simulink model "s_b16a4x512f"  (R2016b)
settings: Solver=VariableStepDiscrete  StartTime=0.0  StopTime=1  RelTol=1e-3
undefined symbols (not defined in the file): fft_stages, n_bits_ants, n_bits_xengs
libraries: xbsIndex_r4 x23057, casper_library_misc x150, xbsReplacements_r4 x9, casper_library_delays x8, xps_library x3
(part 31 of 210)

== system s_b16a4x512f/sys2/pack_out_skarab ==
  note: we must create a gap
      | between packets from
      | mutliple x-engines to allow
      | the buffers on the output switch
      | ports to drain and NIC card
      | to service the packets.
  note: if we become misaligned,
      | then we must flush the buffers
      | by reading one word, waiting "fifo_latency" clocks,
      | then reading another word until we get rb_done.
  note: the last packet
      | might be shorter!
  data_in : Inport
  valid_in : Inport  Port=2
  pkt_rdy : Inport  Port=3
  rb_done : Inport  Port=4
  timestamp : Inport  Port=5
  xeng_id : Inport  Port=6
  go : Inport  Port=7
  gap_size : Inport  Port=8
  AddSub1 : xbsIndex_r4/AddSub  mode=Subtraction  use_carryin=off  use_carryout=off  en=off  latency=1  precision=User Defined  arith_type=Unsigned  n_bits=vector_bits+1  bin_pt=0  quantization=Truncate  overflow=Saturate  use_behavioral_HDL=on  hw_selection=Fabric  pipelined=off  dbl_ovrd=off  block_type=addsub
  Concat : xbsIndex_r4/Concat  num_inputs=2  dbl_ovrd=off  block_type=concat
  Constant : xbsIndex_r4/Constant  const=0  gui_display_data_type=Boolean  arith_type=Boolean  n_bits=16  bin_pt=14  preci_type=Single  exp_width=8  frac_width=24  explicit_period=on  period=1  equ=P=C  opselect=C  inp2=PCIN>>17  opr=+  inp1=P  carry=CIN  dbl_ovrd=off  block_type=constant
  Constant1 : xbsIndex_r4/Constant  const=0  gui_display_data_type=Fixed-point  arith_type=Unsigned  n_bits=spead_lsw  bin_pt=0  preci_type=Single  exp_width=8  frac_width=24  explicit_period=on  period=1  equ=P=C  opselect=C  inp2=PCIN>>17  opr=+  inp1=P  carry=CIN  dbl_ovrd=off  block_type=constant
  Constant15 : xbsIndex_r4/Constant  const=pkt_len  gui_display_data_type=Fixed-point  arith_type=Unsigned  n_bits=vector_bits+1  bin_pt=0  preci_type=Single  exp_width=8  frac_width=24  explicit_period=on  period=1  equ=P=C  opselect=C  inp2=PCIN>>17  opr=+  inp1=P  carry=CIN  dbl_ovrd=off  block_type=constant
  Constant2 : xbsIndex_r4/Constant  const=(vector_len)-1  gui_display_data_type=Fixed-point  arith_type=Unsigned  n_bits=vector_bits+1  bin_pt=0  preci_type=Single  exp_width=8  frac_width=24  explicit_period=on  period=1  equ=P=C  opselect=C  inp2=PCIN>>17  opr=+  inp1=P  carry=CIN  dbl_ovrd=off  block_type=constant
  Constant3 : xbsIndex_r4/Constant  const=vector_len  gui_display_data_type=Fixed-point  arith_type=Unsigned  n_bits=vector_bits+1  bin_pt=0  preci_type=Single  exp_width=8  frac_width=24  explicit_period=on  period=1  equ=P=C  opselect=C  inp2=PCIN>>17  opr=+  inp1=P  carry=CIN  dbl_ovrd=off  block_type=constant
  Constant4 : xbsIndex_r4/Constant  const=0  gui_display_data_type=Boolean  arith_type=Boolean  n_bits=16  bin_pt=14  preci_type=Single  exp_width=8  frac_width=24  explicit_period=on  period=1  equ=P=C  opselect=C  inp2=PCIN>>17  opr=+  inp1=P  carry=CIN  dbl_ovrd=off  block_type=constant
  Constant6 : xbsIndex_r4/Constant  const=heap_len  gui_display_data_type=Fixed-point  arith_type=Unsigned  n_bits=spead_lsw  bin_pt=0  preci_type=Single  exp_width=8  frac_width=24  explicit_period=on  period=1  equ=P=C  opselect=C  inp2=PCIN>>17  opr=+  inp1=P  carry=CIN  dbl_ovrd=off  block_type=constant
  Constant7 : xbsIndex_r4/Constant  const=pkt_len-1  gui_display_data_type=Fixed-point  arith_type=Unsigned  n_bits=pkt_bits  bin_pt=0  preci_type=Single  exp_width=8  frac_width=24  explicit_period=on  period=1  equ=P=C  opselect=C  inp2=PCIN>>17  opr=+  inp1=P  carry=CIN  dbl_ovrd=off  block_type=constant
  Constant8 : xbsIndex_r4/Constant  const=1  gui_display_data_type=Fixed-point  arith_type=Unsigned  n_bits=ceil(log2(fifo_latency))+1  bin_pt=0  preci_type=Single  exp_width=8  frac_width=24  explicit_period=on  period=1  equ=P=C  opselect=C  inp2=PCIN>>17  opr=+  inp1=P  carry=CIN  dbl_ovrd=off  block_type=constant
  Convert{,1..4,6} (6 alike) : xbsIndex_r4/Convert  gui_display_data_type=Fixed-point  arith_type=Unsigned  n_bits=spead_lsw  bin_pt=0  float_type=Single  exp_bits=8  fraction_bits=24  quantization=Truncate  overflow=Wrap  en=off  latency=0  pipeline=off  dbl_ovrd=off  block_type=convert
      settings: block_version=11.4
  Counter1 : xbsIndex_r4/Counter  cnt_type=Free Running  cnt_to=1023  operation=Up  start_count=0  cnt_by_val=1  arith_type=Unsigned  n_bits=vector_bits+1  bin_pt=0  load_pin=off  rst=on  en=on  explicit_period=on  period=1  use_behavioral_HDL=off  implementation=Fabric  use_rpm=on  dbl_ovrd=off  block_type=counter
      settings: xl_area=[0, 0, 0, 0, 0, 0, 0]
  Delay{,3,10..17} (10 alike) : xbsIndex_r4/Delay  rst=off  infoeditControl=Selection of Reset will increase slice count due to use of real FFs and instead of SRLs  en=off  latency=1  reg_retiming=on  dbl_ovrd=off  block_type=delay
      settings: block_version=11.4
  Delay1 : xbsIndex_r4/Delay  rst=off  infoeditControl=Selection of Reset will increase slice count due to use of real FFs and instead of SRLs  en=on  latency=1  reg_retiming=on  dbl_ovrd=off  block_type=delay
  Delay2 : xbsIndex_r4/Delay  rst=off  infoeditControl=Selection of Reset will increase slice count due to use of real FFs and instead of SRLs  en=off  latency=fifo_latency  reg_retiming=on  dbl_ovrd=off  block_type=delay
      settings: block_version=11.4
  Delay4 : xbsIndex_r4/Delay  rst=off  infoeditControl=Selection of Reset will increase slice count due to use of real FFs and instead of SRLs  en=off  latency=fifo_latency  reg_retiming=on  dbl_ovrd=off  block_type=delay
      settings: block_version=11.4
  Delay5 : xbsIndex_r4/Delay  rst=off  infoeditControl=Selection of Reset will increase slice count due to use of real FFs and instead of SRLs  en=on  latency=1  reg_retiming=on  dbl_ovrd=off  block_type=delay
  Delay7 : xbsIndex_r4/Delay  rst=on  infoeditControl=Selection of Reset will increase slice count due to use of real FFs and instead of SRLs  en=on  latency=1  reg_retiming=on  dbl_ovrd=off  block_type=delay
  Delay8 : xbsIndex_r4/Delay  rst=on  infoeditControl=Selection of Reset will increase slice count due to use of real FFs and instead of SRLs  en=on  latency=1  reg_retiming=on  dbl_ovrd=off  block_type=delay
  Delay9 : xbsIndex_r4/Delay  rst=on  infoeditControl=Selection of Reset will increase slice count due to use of real FFs and instead of SRLs  en=on  latency=1  reg_retiming=on  dbl_ovrd=off  block_type=delay
  Gateway Out{1..21} (21 alike) : xbsIndex_r4/Gateway Out  inherit_from_input=off  hdl_port=off  rows=1  columns=1  UseAsDAC=off  DACChannel='1'  interface=None  automatic_assignment=on  address_offset=hex2dec('00')  intf_name=''  intf_description=''  timing_constraint=None  locs_specified=off  LOCs={}  io_standard={}  block_type=gatewayout
      settings: xl_area=[0, 0, 0, 0, 0, 0, 0]  block_version=10.1.3
  Inverter{1..4} (4 alike) : xbsIndex_r4/Inverter  en=off  latency=0  dbl_ovrd=off  block_type=inv
      settings: block_version=11.4
  Logical{1,3..5,13..14} (6 alike) : xbsIndex_r4/Logical  logical_function=OR  inputs=2  en=off  latency=0  precision=Full  arith_type=Unsigned  n_bits=8  bin_pt=2  align_bp=on  dbl_ovrd=off  block_type=logical
      settings: xl_area=[0, 0, 0, 0, 0, 0, 0]
  Logical{2,8..12,15} (7 alike) : xbsIndex_r4/Logical  logical_function=AND  inputs=2  en=off  latency=0  precision=Full  arith_type=Unsigned  n_bits=8  bin_pt=2  align_bp=on  dbl_ovrd=off  block_type=logical
      settings: xl_area=[0, 0, 0, 0, 0, 0, 0]
  Logical6 : xbsIndex_r4/Logical  logical_function=AND  inputs=2  en=off  latency=1  precision=Full  arith_type=Unsigned  n_bits=8  bin_pt=2  align_bp=on  dbl_ovrd=off  block_type=logical
      settings: xl_area=[0, 0, 0, 0, 0, 0, 0]
  Logical7 : xbsIndex_r4/Logical  logical_function=XOR  inputs=2  en=off  latency=0  precision=Full  arith_type=Unsigned  n_bits=8  bin_pt=2  align_bp=on  dbl_ovrd=off  block_type=logical
      settings: xl_area=[0, 0, 0, 0, 0, 0, 0]
  Mux1 : xbsIndex_r4/Mux  inputs=2  en=off  latency=1  precision=Full  arith_type="Signed  (2's comp)"  n_bits=8  bin_pt=2  quantization=Truncate  overflow=Wrap  dbl_ovrd=off  block_type=mux
      settings: xl_area=[0, 0, 0, 0, 0, 0, 0]
  Reinterpret : xbsIndex_r4/Reinterpret  force_arith_type=on  arith_type=Unsigned  force_bin_pt=on  bin_pt=0  block_type=reinterpret
      settings: infoedit="Changes signal type without altering the binary representation.   You can changed the signal between signed and unsigned, and relocate the binary point.<br><br>Hardware notes: In hardware this block costs nothing.<br><br>Example:  Suppose the input is 6 bits wide, signed, with 2 fractional bits, and the output is forced to unsigned with 0 fractional bits.  Then an input of -2.0 (1110.00 in binary 2's complement) becomes an output of 56 (111000 in binary)."
  Relational1 : xbsIndex_r4/Relational  mode=a=b  op_type=Bool  en=off  latency=0  dbl_ovrd=off  block_type=relational
      settings: xl_area=[0, 0, 0, 0, 0, 0, 0]  block_version=10.1.3
  Relational2 : xbsIndex_r4/Relational  mode=a<b  op_type=Bool  en=off  latency=0  dbl_ovrd=off  block_type=relational
      settings: xl_area=[0, 0, 0, 0, 0, 0, 0]  block_version=10.1.3
  Relational4 : xbsIndex_r4/Relational  mode=a=b  op_type=Bool  en=off  latency=0  dbl_ovrd=off  block_type=relational
      settings: xl_area=[0, 0, 0, 0, 0, 0, 0]  block_version=10.1.3
  Relational5 : xbsIndex_r4/Relational  mode=a=b  op_type=Bool  en=off  latency=0  dbl_ovrd=off  block_type=relational
      settings: xl_area=[0, 0, 0, 0, 0, 0, 0]  block_version=10.1.3
  Shift1 : xbsIndex_r4/Shift  shift_dir=Left  shift_bits=n_bits_word_size  en=off  latency=0  precision=Full  arith_type="Signed  (2's comp)"  n_bits=16  bin_pt=14  quantization=Truncate  overflow=Wrap  dbl_ovrd=off  block_type=shift
  Shift2 : xbsIndex_r4/Shift  shift_dir=Left  shift_bits=n_bits_chans  en=off  latency=0  precision=Full  arith_type="Signed  (2's comp)"  n_bits=16  bin_pt=14  quantization=Truncate  overflow=Wrap  dbl_ovrd=off  block_type=shift
  Slice : xbsIndex_r4/Slice  nbits=pkt_bits  boolean_output=off  mode=Lower Bit Location + Width  bit1=0  base1=MSB of Input  bit0=0  base0=LSB of Input  dbl_ovrd=off  block_type=slice
  Slice1 : xbsIndex_r4/Slice  nbits=1  boolean_output=off  mode=Two Bit Locations  bit1=0  base1=MSB of Input  bit0=n_bits_timestamp_padding  base0=LSB of Input  dbl_ovrd=off  block_type=slice
  edge_detect : Subsystem  AncestorBlock=casper_library_misc/edge_detect  mask(edge_detect){edge=Rising, polarity=Active High, x_in=[0 0.08 0.08 0.16 0.16 0.24 0.24 0.32 0.32 0.4], y_in=[-1 -1  1  1  1  1  1  1  1  1], x_out=[0.6 0.68 0.68 0.76 0.76 0.84 0.84 0.92 0.92 1], y_out=[-1 -1  1  1 -1 -1 -1 -1 -1 -1]}
      mask prompts: edge "Edge Type"; polarity "Output Polarity"; x_in "Input X Positions"; y_in "Input Y Positions"; x_out "Output X Positions"; y_out "Output Y Positions"
      mask help: Output is active for one-cycle after each edge of the specified type (i.e. rising, falling or both).
      mask init: same as s_b16a4x512f/edge_detect
      settings: AttributesFormatString=|
      | rising edges
      | active high
      mask Help: Output is active for one-cycle after each edge of the specified type (i.e. rising, falling, or both).  Latency is zero.
      mask TypeOptions edge: Rising | Falling | Both
      mask TypeOptions polarity: Active High | Active Low
      mask Display:
      | plot(x_in_num,0.5+y_in_num*0.2);
      | plot(x_out_num,0.5+y_out_num*0.2);
  edge_detect1 : Subsystem  AncestorBlock=casper_library_misc/edge_detect  mask(edge_detect){edge=Rising, polarity=Active High, x_in=[0 0.08 0.08 0.16 0.16 0.24 0.24 0.32 0.32 0.4], y_in=[-1 -1  1  1  1  1  1  1  1  1], x_out=[0.6 0.68 0.68 0.76 0.76 0.84 0.84 0.92 0.92 1], y_out=[-1 -1  1  1 -1 -1 -1 -1 -1 -1]}
      mask prompts: edge "Edge Type"; polarity "Output Polarity"; x_in "Input X Positions"; y_in "Input Y Positions"; x_out "Output X Positions"; y_out "Output Y Positions"
      mask help: Output is active for one-cycle after each edge of the specified type (i.e. rising, falling or both).
      mask init: same as s_b16a4x512f/edge_detect
      settings: AttributesFormatString=|
      | rising edges
      | active high
      mask Help: Output is active for one-cycle after each edge of the specified type (i.e. rising, falling, or both).  Latency is zero.
      mask TypeOptions edge: Rising | Falling | Both
      mask TypeOptions polarity: Active High | Active Low
      mask Display:
      | plot(x_in_num,0.5+y_in_num*0.2);
      | plot(x_out_num,0.5+y_out_num*0.2);
  edge_detect2 : Subsystem  AncestorBlock=casper_library_misc/edge_detect  mask(edge_detect){edge=Rising, polarity=Active High, x_in=[0 0.08 0.08 0.16 0.16 0.24 0.24 0.32 0.32 0.4], y_in=[-1 -1  1  1  1  1  1  1  1  1], x_out=[0.6 0.68 0.68 0.76 0.76 0.84 0.84 0.92 0.92 1], y_out=[-1 -1  1  1 -1 -1 -1 -1 -1 -1]}
      mask prompts: edge "Edge Type"; polarity "Output Polarity"; x_in "Input X Positions"; y_in "Input Y Positions"; x_out "Output X Positions"; y_out "Output Y Positions"
      mask help: Output is active for one-cycle after each edge of the specified type (i.e. rising, falling or both).
      mask init: same as s_b16a4x512f/edge_detect
      settings: AttributesFormatString=|
      | rising edges
      | active high
      mask Help: Output is active for one-cycle after each edge of the specified type (i.e. rising, falling, or both).  Latency is zero.
      mask TypeOptions edge: Rising | Falling | Both
      mask TypeOptions polarity: Active High | Active Low
      mask Display:
      | plot(x_in_num,0.5+y_in_num*0.2);
      | plot(x_out_num,0.5+y_out_num*0.2);
  edge_detect3 : Subsystem  AncestorBlock=casper_library_misc/edge_detect  mask(edge_detect){edge=Rising, polarity=Active High, x_in=[0 0.08 0.08 0.16 0.16 0.24 0.24 0.32 0.32 0.4], y_in=[-1 -1  1  1  1  1  1  1  1  1], x_out=[0.6 0.68 0.68 0.76 0.76 0.84 0.84 0.92 0.92 1], y_out=[-1 -1  1  1 -1 -1 -1 -1 -1 -1]}
      mask prompts: edge "Edge Type"; polarity "Output Polarity"; x_in "Input X Positions"; y_in "Input Y Positions"; x_out "Output X Positions"; y_out "Output Y Positions"
      mask help: Output is active for one-cycle after each edge of the specified type (i.e. rising, falling or both).
      mask init: same as s_b16a4x512f/edge_detect
      settings: AttributesFormatString=|
      | rising edges
      | active high
      mask Help: Output is active for one-cycle after each edge of the specified type (i.e. rising, falling, or both).  Latency is zero.
      mask TypeOptions edge: Rising | Falling | Both
      mask TypeOptions polarity: Active High | Active Low
      mask Display:
      | plot(x_in_num,0.5+y_in_num*0.2);
      | plot(x_out_num,0.5+y_out_num*0.2);
  edge_detect4 : Subsystem  AncestorBlock=casper_library_misc/edge_detect  mask(edge_detect){edge=Rising, polarity=Active High, x_in=[0 0.08 0.08 0.16 0.16 0.24 0.24 0.32 0.32 0.4], y_in=[-1 -1  1  1  1  1  1  1  1  1], x_out=[0.6 0.68 0.68 0.76 0.76 0.84 0.84 0.92 0.92 1], y_out=[-1 -1  1  1 -1 -1 -1 -1 -1 -1]}
      mask prompts: edge "Edge Type"; polarity "Output Polarity"; x_in "Input X Positions"; y_in "Input Y Positions"; x_out "Output X Positions"; y_out "Output Y Positions"
      mask help: Output is active for one-cycle after each edge of the specified type (i.e. rising, falling or both).
      mask init: same as s_b16a4x512f/edge_detect
      settings: AttributesFormatString=|
      | rising edges
      | active high
      mask Help: Output is active for one-cycle after each edge of the specified type (i.e. rising, falling, or both).  Latency is zero.
      mask TypeOptions edge: Rising | Falling | Both
      mask TypeOptions polarity: Active High | Active Low
      mask Display:
      | plot(x_in_num,0.5+y_in_num*0.2);
      | plot(x_out_num,0.5+y_out_num*0.2);
  gap_creator : xbsIndex_r4/Counter  cnt_type=Free Running  cnt_to=Inf  operation=Up  start_count=0  cnt_by_val=1  arith_type=Unsigned  n_bits=n_bits_max_gap  bin_pt=0  load_pin=off  rst=on  en=on  explicit_period=on  period=1  use_behavioral_HDL=off  implementation=Fabric  dbl_ovrd=off  block_type=counter
  gap_done : xbsIndex_r4/Relational  mode=a<b  op_type=Bool  en=off  latency=1  dbl_ovrd=off  block_type=relational
  hdr_check : Scope  NumInputPorts=5
  hdr_check1 : Scope  NumInputPorts=5
  pack_xeng : Subsystem  Tag=casper:spead_pack  AncestorBlock=casper_library_communications/spead_pack  mask(pkt_pack_mask){max_pkt_len_bits=8, header_ids=0x1600, 0x4103, header_ind_ids=0x1800, spead_msw=64, spead_lsw=48, spead_version=4, bytes_per_word=8}
      mask prompts: max_pkt_len_bits "Max pkt length, 2^? 64-bit words"; header_ids "SPEAD direct address IDs (decimal)"; header_ind_ids "SPEAD indirect address IDs (decimal)"; spead_msw "SPEAD Flavour (MSw)"; spead_lsw "SPEAD Flavour (LSw)"; spead_version "SPEAD version"; bytes_per_word "Word size, in bytes"
      mask help:
      | This block generates SPEAD-compliant packets from a datastream.
      |
      | Packets are created with a fixed header followed by a number of 64-bit items.
      |
      | Requires a 64-bit data stream.
      |
      | The data_ready signal is one cycle BEFORE valid data! Does not have to be with a valid signal either.
      mask init:
      | % if floor(log2(bytes_per_word)) ~= log2(bytes_per_word)
      | %     error('Bytes per word should be a power of two.');
      | % end
      | % 
      | % spead_pack_init(gcb)
  packetise_output : Scope  NumInputPorts=11
  payload_cnt4 : xbsIndex_r4/Counter  cnt_type=Count Limited  cnt_to=max((fifo_latency + 1),2)  operation=Up  start_count=0  cnt_by_val=1  arith_type=Unsigned  n_bits=ceil(log2(fifo_latency))+1  bin_pt=0  load_pin=off  rst=on  en=on  explicit_period=on  period=1  use_behavioral_HDL=off  implementation=Fabric  use_rpm=on  dbl_ovrd=off  block_type=counter
      settings: xl_area=[0, 0, 0, 0, 0, 0, 0]
  data_out : Outport
  valid_out : Outport  Port=2
  eof : Outport  Port=3
  err : Outport  Port=4
  fetch : Outport  Port=5
  pkt_ready : Outport  Port=6
  wires:
  edge_detect4/1(out) -> gap_creator/1
  Convert6/1 -> Shift2/1
  Constant1/1 -> pack_xeng/10(hdr8_0x1800)
  Convert2/1 -> [heap_cnt]
  Concat/1 -> Convert2/1
  [xeng_id] -> Concat/2
  Slice1/1 -> Concat/1
  [timestamp] -> Slice1/1
  gap_size/1 -> [gap_size]
  Delay13/1 -> pack_xeng/9(hdr6_0x4103_DIR)
  [freq_offset] -> Delay13/1
  Shift2/1 -> [freq_offset]
  [xeng_id] -> Convert6/1
  Convert4/1 -> Delay16/1
  [gap_size] -> gap_done/2
  pack_xeng/3(eof) -> Logical3/1
  Logical3/1 -> eof/1
  Gateway Out15/1 -> packetise_output/7
  [end_of_vector] -> Logical5/1
  Gateway Out9/1 -> packetise_output/6
  Gateway Out14/1 -> packetise_output/5
  Gateway Out6/1 -> packetise_output/4
  Gateway Out8/1 -> packetise_output/3
  Gateway Out1/1 -> packetise_output/2
  Gateway Out7/1 -> packetise_output/1
  Logical5/1 -> [eof]
  Logical2/1 -> [rb_done]
  xeng_id/1 -> [xeng_id]
  Reinterpret/1 -> [data_input]
  Gateway Out11/1 -> packetise_output/8
  Slice/1 -> Relational1/1
  Counter1/1 -> [vector_position], Slice/1, Relational5/1
  timestamp/1 -> Delay5/1
  Delay5/1 -> [timestamp]
  [vector_start] -> Delay5/2
  Constant2/1 -> Relational5/2
  Relational5/1 -> [end_of_vector]
  data_in/1 -> Reinterpret/1, [raw_data_input]
  valid_in/1 -> Logical2/1, [valid_input]
  pkt_rdy/1 -> [pkt_rdy]
  rb_done/1 -> Logical2/2
  Gateway Out18/1 -> packetise_output/9
  Gateway Out17/1 -> packetise_output/10
  [valid_input] -> [valid_output]
  [fetch_pld] -> Counter1/2
  [vector_start] -> Counter1/1
  Constant7/1 -> Relational1/2
  Relational1/1 -> Logical5/2
  [fetch_pld] -> Gateway Out6/1
  [busy] -> Gateway Out15/1
  [valid_output] -> Gateway Out1/1
  [busy_pkt] -> Gateway Out9/1
  [raw_data_input] -> Gateway Out7/1
  [vector_position] -> Gateway Out11/1
  pack_xeng/1(data_out) -> data_out/1, [data_out]
  [vector_position] -> Delay1/1
  Delay1/1 -> AddSub1/2, Delay17/1
  [get_a_pkt] -> Delay1/2
  [rb_done] -> Logical7/1
  [end_of_vector] -> Delay2/1
  Delay17/1 -> Convert/1
  Convert/1 -> Shift1/1
  [vector_start] -> Logical4/1
  Logical4/1 -> Delay4/1
  [go] -> Logical8/1
  Logical8/1 -> Delay3/1
  Delay7/1 -> [busy], edge_detect/1(in)
  edge_detect/1(out) -> [vector_start]
  Inverter2/1 -> Logical10/1
  Logical10/1 -> Delay7/1, Delay7/3
  [end_of_vector] -> Logical1/2
  [go] -> Delay/1
  edge_detect1/1(out) -> Logical10/2
  [busy] -> Inverter2/1
  Delay/1 -> edge_detect1/1(in)
  Delay2/1 -> Logical7/2
  [get_a_pkt] -> Inverter1/1
  Delay3/1 -> Logical4/2
  Delay4/1 -> Delay8/1, Delay8/3
  edge_detect2/1(out) -> [get_a_pkt]
  Delay8/1 -> [busy_pkt], edge_detect2/1(in)
  [eof] -> Delay8/2
  [busy] -> Logical8/2
  Inverter1/1 -> Logical9/1
  Logical9/1 -> [fetch_pld]
  [eof] -> Gateway Out18/1
  [pkt_rdy] -> Gateway Out17/1
  Logical7/1 -> Delay9/1, Delay9/3, [err]
  [rb_done] -> Logical12/2
  payload_cnt4/1 -> Relational4/2
  Constant8/1 -> Relational4/1
  Delay9/1 -> payload_cnt4/2, [flushing]
  Relational4/1 -> [stutter_flush]
  Logical1/1 -> Delay7/2
  [err] -> Logical1/1
  [valid_output] -> Logical11/1
  Inverter3/1 -> Logical11/2, Logical15/2
  [flushing] -> Inverter3/1
  Logical12/1 -> Delay9/2, payload_cnt4/1
  [flushing] -> Logical12/1
  Logical13/1 -> fetch/1
  [fetch_pld] -> Logical13/1
  [stutter_flush] -> Logical13/2
  [data_out] -> Gateway Out2/1
  [vector_start] -> Gateway Out3/1
  [heap_cnt] -> Gateway Out4/1
  [heap_offset] -> Gateway Out5/1
  Gateway Out2/1 -> hdr_check/1
  Gateway Out3/1 -> hdr_check/2
  Gateway Out4/1 -> hdr_check/3
  Gateway Out5/1 -> hdr_check/4
  Constant15/1 -> Relational2/2, Mux1/2
  Mux1/1 -> Convert1/1
  Relational2/1 -> Mux1/1
  Constant3/1 -> AddSub1/1
  AddSub1/1 -> Mux1/3, Relational2/1
  Convert1/1 -> [pld_len]
  Shift1/1 -> [heap_offset]
  Gateway Out10/1 -> hdr_check/5
  [pld_len] -> Gateway Out10/1
  gap_creator/1 -> gap_done/1, [gap_count]
  go/1 -> [go]
  gap_done/1 -> Inverter4/1, gap_creator/2
  Inverter4/1 -> Logical6/1
  [pkt_rdy] -> Logical6/2
  Logical6/1 -> pkt_ready/1
  [eof] -> edge_detect4/1(in)
  Gateway Out16/1 -> packetise_output/11
  [gap_count] -> Gateway Out16/1
  [data_input] -> Delay11/1
  [heap_cnt] -> Convert3/1
  [heap_offset] -> Delay14/1
  Logical11/1 -> Delay10/1
  pack_xeng/2(valid_out) -> valid_out/1
  [pld_len] -> Delay15/1
  Logical14/1 -> Logical3/2, err/1
  pack_xeng/4(data_overflow) -> [data_overflow], Logical14/2
  [err] -> Logical14/1
  [valid_output] -> Logical15/1
  edge_detect3/1(out) -> pack_xeng/1(data256_ready)
  Logical15/1 -> edge_detect3/1(in)
  Delay10/1 -> pack_xeng/2(data256_valid)
  Delay11/1 -> pack_xeng/3(data256)
  Delay12/1 -> pack_xeng/4(hdr_heap_id)
  Constant6/1 -> pack_xeng/5(hdr_heap_size)
  Delay14/1 -> pack_xeng/6(hdr_heap_offset)
  Delay15/1 -> pack_xeng/7(hdr_pkt_len_words)
  Delay16/1 -> pack_xeng/8(hdr5_0x1600_DIR)
  Gateway Out20/1 -> hdr_check1/4
  Gateway Out12/1 -> hdr_check1/1
  Gateway Out19/1 -> hdr_check1/3
  Gateway Out21/1 -> hdr_check1/5
  Gateway Out13/1 -> hdr_check1/2
  [valid_input] -> Gateway Out12/1
  [rb_done] -> Gateway Out13/1
  [end_of_vector] -> Gateway Out19/1
  [err] -> Gateway Out20/1
  [data_overflow] -> Gateway Out21/1
  [busy_pkt] -> Logical9/2
  Constant/1 -> Gateway Out8/1
  Constant4/1 -> Gateway Out14/1
  Convert3/1 -> Delay12/1
  [timestamp] -> Convert4/1

== system s_b16a4x512f/sys2/pipeline ==
  d : Inport
  Register0 : xbsIndex_r4/Register  init=0  rst=off  en=off  dbl_ovrd=off  block_type=register
      settings: block_version=11.4
  Register1 : xbsIndex_r4/Register  init=0  rst=off  en=off  dbl_ovrd=off  block_type=register
      settings: block_version=11.4
  q : Outport
  wires:
  Register0/1 -> Register1/1
  d/1 -> Register0/1
  Register1/1 -> q/1

== system s_b16a4x512f/sys2/pipeline1 ==
  d : Inport
  Register0 : xbsIndex_r4/Register  init=0  rst=off  en=off  dbl_ovrd=off  block_type=register
      settings: block_version=11.4
  Register1 : xbsIndex_r4/Register  init=0  rst=off  en=off  dbl_ovrd=off  block_type=register
      settings: block_version=11.4
  q : Outport
  wires:
  Register1/1 -> q/1
  d/1 -> Register0/1
  Register0/1 -> Register1/1

== system s_b16a4x512f/sys2/pipeline10 ==
  d : Inport
  Register0 : xbsIndex_r4/Register  init=0  rst=off  en=off  dbl_ovrd=off  block_type=register
      settings: block_version=11.4
  Register1 : xbsIndex_r4/Register  init=0  rst=off  en=off  dbl_ovrd=off  block_type=register
      settings: block_version=11.4
  q : Outport
  wires:
  Register0/1 -> Register1/1
  d/1 -> Register0/1
  Register1/1 -> q/1

== system s_b16a4x512f/sys2/pipeline11 ==
  d : Inport
  Register0 : xbsIndex_r4/Register  init=0  rst=off  en=off  dbl_ovrd=off  block_type=register
      settings: block_version=11.4
  Register1 : xbsIndex_r4/Register  init=0  rst=off  en=off  dbl_ovrd=off  block_type=register
      settings: block_version=11.4
  q : Outport
  wires:
  Register1/1 -> q/1
  d/1 -> Register0/1
  Register0/1 -> Register1/1

== system s_b16a4x512f/sys2/pipeline12 ==
  d : Inport
  Register0 : xbsIndex_r4/Register  init=0  rst=off  en=off  dbl_ovrd=off  block_type=register
      settings: block_version=11.4
  Register1 : xbsIndex_r4/Register  init=0  rst=off  en=off  dbl_ovrd=off  block_type=register
      settings: block_version=11.4
  q : Outport
  wires:
  Register0/1 -> Register1/1
  d/1 -> Register0/1
  Register1/1 -> q/1

== system s_b16a4x512f/sys2/pipeline13 ==
  d : Inport
  Register0 : xbsIndex_r4/Register  init=0  rst=off  en=off  dbl_ovrd=off  block_type=register
      settings: block_version=11.4
  Register1 : xbsIndex_r4/Register  init=0  rst=off  en=off  dbl_ovrd=off  block_type=register
      settings: block_version=11.4
  q : Outport
  wires:
  Register1/1 -> q/1
  d/1 -> Register0/1
  Register0/1 -> Register1/1

== system s_b16a4x512f/sys2/pipeline2 ==
  d : Inport
  Register0 : xbsIndex_r4/Register  init=0  rst=off  en=off  dbl_ovrd=off  block_type=register
      settings: block_version=11.4
  Register1 : xbsIndex_r4/Register  init=0  rst=off  en=off  dbl_ovrd=off  block_type=register
      settings: block_version=11.4
  q : Outport
  wires:
  Register0/1 -> Register1/1
  d/1 -> Register0/1
  Register1/1 -> q/1

== system s_b16a4x512f/sys2/pipeline3 ==
  d : Inport
  Register0 : xbsIndex_r4/Register  init=0  rst=off  en=off  dbl_ovrd=off  block_type=register
      settings: block_version=11.4
  Register1 : xbsIndex_r4/Register  init=0  rst=off  en=off  dbl_ovrd=off  block_type=register
      settings: block_version=11.4
  q : Outport
  wires:
  Register1/1 -> q/1
  d/1 -> Register0/1
  Register0/1 -> Register1/1

== system s_b16a4x512f/sys2/pipeline4 ==
  d : Inport
  Register0 : xbsIndex_r4/Register  init=0  rst=off  en=off  dbl_ovrd=off  block_type=register
      settings: block_version=11.4
  Register1 : xbsIndex_r4/Register  init=0  rst=off  en=off  dbl_ovrd=off  block_type=register
      settings: block_version=11.4
  q : Outport
  wires:
  Register1/1 -> q/1
  d/1 -> Register0/1
  Register0/1 -> Register1/1

== system s_b16a4x512f/sys2/pipeline5 ==
  d : Inport
  Register0 : xbsIndex_r4/Register  init=0  rst=off  en=off  dbl_ovrd=off  block_type=register
      settings: block_version=11.4
  Register1 : xbsIndex_r4/Register  init=0  rst=off  en=off  dbl_ovrd=off  block_type=register
      settings: block_version=11.4
  q : Outport
  wires:
  Register0/1 -> Register1/1
  d/1 -> Register0/1
  Register1/1 -> q/1

== system s_b16a4x512f/sys2/pipeline6 ==
  d : Inport
  Register0 : xbsIndex_r4/Register  init=0  rst=off  en=off  dbl_ovrd=off  block_type=register
      settings: block_version=11.4
  Register1 : xbsIndex_r4/Register  init=0  rst=off  en=off  dbl_ovrd=off  block_type=register
      settings: block_version=11.4
  q : Outport
  wires:
  Register1/1 -> q/1
  d/1 -> Register0/1
  Register0/1 -> Register1/1

== system s_b16a4x512f/sys2/pipeline7 ==
  d : Inport
  Register0 : xbsIndex_r4/Register  init=0  rst=off  en=off  dbl_ovrd=off  block_type=register
      settings: block_version=11.4
  Register1 : xbsIndex_r4/Register  init=0  rst=off  en=off  dbl_ovrd=off  block_type=register
      settings: block_version=11.4
  q : Outport
  wires:
  Register0/1 -> Register1/1
  d/1 -> Register0/1
  Register1/1 -> q/1

== system s_b16a4x512f/sys2/pipeline8 ==
  d : Inport
  Register0 : xbsIndex_r4/Register  init=0  rst=off  en=off  dbl_ovrd=off  block_type=register
      settings: block_version=11.4
  Register1 : xbsIndex_r4/Register  init=0  rst=off  en=off  dbl_ovrd=off  block_type=register
      settings: block_version=11.4
  q : Outport
  wires:
  Register0/1 -> Register1/1
  d/1 -> Register0/1
  Register1/1 -> q/1

== system s_b16a4x512f/sys2/pipeline9 ==
  d : Inport
  Register0 : xbsIndex_r4/Register  init=0  rst=off  en=off  dbl_ovrd=off  block_type=register
      settings: block_version=11.4
  Register1 : xbsIndex_r4/Register  init=0  rst=off  en=off  dbl_ovrd=off  block_type=register
      settings: block_version=11.4
  q : Outport
  wires:
  Register0/1 -> Register1/1
  d/1 -> Register0/1
  Register1/1 -> q/1

== system s_b16a4x512f/sys2/pkt_reord ==
  note: While reading a window out,
      | we erase the contents of that window,
      | and set the MSb (comms error).
  note: BRAM depth is
      | X int length * # antennas * # windows
  din : Inport
  valid_in : Inport  Port=2
  pkt_idx : Inport  Port=3
  time : Inport  Port=4
  ant : Inport  Port=5
  freq : Inport  Port=6
  board_id : Inport  Port=7
  Concat : xbsIndex_r4/Concat  num_inputs=2  dbl_ovrd=off  block_type=concat
  Concat1 : xbsIndex_r4/Concat  num_inputs=2  dbl_ovrd=off  block_type=concat
  Concat2 : xbsIndex_r4/Concat  num_inputs=2  dbl_ovrd=off  block_type=concat
  Constant : xbsIndex_r4/Constant  const=0  gui_display_data_type=Fixed-point  arith_type=Unsigned  n_bits=1  bin_pt=0  preci_type=Single  exp_width=8  frac_width=24  explicit_period=on  period=1  equ=P=C  opselect=C  inp2=PCIN>>17  opr=+  inp1=P  carry=CIN  dbl_ovrd=off  block_type=constant
  Constant1 : xbsIndex_r4/Constant  const=2^ant_bits  gui_display_data_type=Fixed-point  arith_type=Unsigned  n_bits=ant_bits+1  bin_pt=0  preci_type=Single  exp_width=8  frac_width=24  explicit_period=on  period=1  equ=P=C  opselect=C  inp2=PCIN>>17  opr=+  inp1=P  carry=CIN  dbl_ovrd=off  block_type=constant
  Constant2 : xbsIndex_r4/Constant  const=1  gui_display_data_type=Fixed-point  arith_type=Unsigned  n_bits=1  bin_pt=0  preci_type=Single  exp_width=8  frac_width=24  explicit_period=on  period=1  equ=P=C  opselect=C  inp2=PCIN>>17  opr=+  inp1=P  carry=CIN  dbl_ovrd=off  block_type=constant
  Constant3 : xbsIndex_r4/Constant  const=2^(x_int_bits-n_bits_input_words)  gui_display_data_type=Fixed-point  arith_type=Unsigned  n_bits=x_int_bits  bin_pt=0  preci_type=Single  exp_width=8  frac_width=24  explicit_period=on  period=1  equ=P=C  opselect=C  inp2=PCIN>>17  opr=+  inp1=P  carry=CIN  dbl_ovrd=off  block_type=constant
  Constant4 : xbsIndex_r4/Constant  const=0  gui_display_data_type=Fixed-point  arith_type=Unsigned  n_bits=n_bits_data  bin_pt=0  preci_type=Single  exp_width=8  frac_width=24  explicit_period=on  period=1  equ=P=C  opselect=C  inp2=PCIN>>17  opr=+  inp1=P  carry=CIN  dbl_ovrd=off  block_type=constant
  Delay1 : xbsIndex_r4/Delay  rst=off  infoeditControl=Selection of Reset will increase slice count due to use of real FFs and instead of SRLs  en=off  latency=3  reg_retiming=on  dbl_ovrd=off  block_type=delay
      settings: infoedit=Hardware notes: A delay line is a chain, each link of which is an SRL16 or SRL32 followed by a flip-flop.  xl_area=[0, 0, 0, 0, 0, 0, 0]
  Delay20 : xbsIndex_r4/Delay  rst=off  infoeditControl=Selection of Reset will increase slice count due to use of real FFs and instead of SRLs  en=off  latency=3  reg_retiming=on  dbl_ovrd=off  block_type=delay
      settings: infoedit=Hardware notes: A delay line is a chain, each link of which is an SRL16 or SRL32 followed by a flip-flop.  xl_area=[0, 0, 0, 0, 0, 0, 0]
  Delay21 : xbsIndex_r4/Delay  rst=off  infoeditControl=Selection of Reset will increase slice count due to use of real FFs and instead of SRLs  en=off  latency=3  reg_retiming=on  dbl_ovrd=off  block_type=delay
      settings: infoedit=Hardware notes: A delay line is a chain, each link of which is an SRL16 or SRL32 followed by a flip-flop.  xl_area=[0, 0, 0, 0, 0, 0, 0]
  Delay23 : xbsIndex_r4/Delay  rst=off  infoeditControl=Selection of Reset will increase slice count due to use of real FFs and instead of SRLs  en=off  latency=2  reg_retiming=on  dbl_ovrd=off  block_type=delay
      settings: xl_area=[0, 0, 0, 0, 0, 0, 0]
  Delay24 : xbsIndex_r4/Delay  rst=off  infoeditControl=Selection of Reset will increase slice count due to use of real FFs and instead of SRLs  en=off  latency=2  reg_retiming=on  dbl_ovrd=off  block_type=delay
      settings: xl_area=[0, 0, 0, 0, 0, 0, 0]
  Delay25 : xbsIndex_r4/Delay  rst=off  infoeditControl=Selection of Reset will increase slice count due to use of real FFs and instead of SRLs  en=off  latency=2  reg_retiming=on  dbl_ovrd=off  block_type=delay
      settings: xl_area=[0, 0, 0, 0, 0, 0, 0]
  Logical : xbsIndex_r4/Logical  logical_function=AND  inputs=2  en=off  latency=0  precision=Full  arith_type=Unsigned  n_bits=16  bin_pt=0  align_bp=on  dbl_ovrd=off  block_type=logical
  Terminator1 : Terminator
  ant_check : xbsIndex_r4/Assert  assert_type=on  type_source=Explicitly  gui_display_data_type=Fixed-point  arith_type=Unsigned  n_bits=ant_bits  bin_pt=0  preci_type=Single  exp_width=8  frac_width=24  assert_rate=off  rate_source=Explicitly  period=1  output_port=on  block_type=assert
  bus_expand : Subsystem  AncestorBlock=casper_library_flow_control/bus_expand  mask(bus_expand){mode=divisions of arbitrary size, outputNum=1, outputWidth=[2^n_bits_output_words, (2^n_bits_output_words)*n_bits_data], outputBinaryPt=[0, 0], outputArithmeticType=[2, 0], show_format=off, outputToWorkspace=off, variablePrefix=out, outputToModelAsWell=on}
      mask prompts: outputNum "Number of outputs:"; outputWidth "Output width [msb ... lsb]:"; outputBinaryPt "Output binary point position [msb ... lsb]:"; outputArithmeticType "Output arithmetic type (ufix=0, fix=1, bool=2) [msb ... lsb]:"; show_format "Print format string?"; outputToWorkspace "Output to workspace?"; variablePrefix "Variable name prefix:"; outputToModelAsWell "Output to model as well?"
      mask help:
      | Expands a 'bus' made using a bus_create or Xilinx
      | concat block.
      | The input will be divided into the specified number
      | of outputs with the specified arithmetic types.
      | Divisions are made from most significant bit.
      mask init: same as s_b16a4x512f/bus_expand
      settings: AttributesFormatString=2 outputs
      mask TypeOptions mode: divisions of equal size | divisions of arbitrary size
      mask Callback mode: bus_expand_callback();
      mask Callback outputWidth: bus_expand_callback();
      mask Callback outputToWorkspace: bus_expand_callback();
  bus_replicate : Subsystem  AncestorBlock=casper_library_bus/bus_replicate  mask(bus_replicate){replication=2^n_bits_output_words, latency=0, misc=off, implementation=behavioral}
      mask prompts: replication "replication factor"; misc "misc support"; implementation "delay implementation"
      mask help: Output bus formed by replicating input bus a number of times
      mask init:
      | bus_replicate_init(gcb, ...
      |     'replication', replication, ...
      |     'latency', latency, ...
      |     'implementation', implementation, ...
      |     'misc', misc);
      mask TypeOptions implementation: core | behavioral
  data_buffer : xbsIndex_r4/Dual Port RAM  depth=2^x_int_bits * 2^ant_bits * 2^window_bits  initVector=zeros(1, 2^x_int_bits * 2^ant_bits * 2^window_bits)  distributed_mem=Block RAM  init_a=0  init_b=0  rst_a=off  rst_b=off  en_a=off  en_b=off  latency=3  write_mode_A=Read Before Write  write_mode_B=Read Before Write  optimize=Speed  dbl_ovrd=off  block_type=dpram
      settings: xl_area=[0, 0, 0, 0, 0, 0, 0]  block_version=10.1.3
  data_check : xbsIndex_r4/Assert  assert_type=on  type_source=Explicitly  gui_display_data_type=Fixed-point  arith_type=Unsigned  n_bits=n_bits_data * 2^n_bits_input_words  bin_pt=0  preci_type=Single  exp_width=8  frac_width=24  assert_rate=off  rate_source=Explicitly  period=1  output_port=on  block_type=assert
  freq_check : xbsIndex_r4/Assert  assert_type=on  type_source=Explicitly  gui_display_data_type=Fixed-point  arith_type=Unsigned  n_bits=chan_bits-xeng_bits  bin_pt=0  preci_type=Single  exp_width=8  frac_width=24  assert_rate=off  rate_source=Explicitly  period=1  output_port=on  block_type=assert
  input_control : Subsystem
  munge : Subsystem  AncestorBlock=casper_library_flow_control/munge  mask(munge){divisions=1 + 2^n_bits_input_words, div_size=[1, repmat(n_bits_data, 1, 2^n_bits_input_words)], order=reshape([zeros(1, 2^n_bits_input_words); (1+2^n_bits_input_words)-(1:2^n_bits_input_words)], 1, 2^(n_bits_input_words+1)), arith_type_out=Unsigned, bin_pt_out=0}
      mask prompts: divisions "Number of divisions"; div_size "Division size (bits)"; order "Division packing order"; arith_type_out "Output arithmetic type"; bin_pt_out "Output binary point"
      mask help: Splits an input bus into the specified number of divisions and then recombines them in the order specified (most significant division = 0,least = number divisions-1)
      mask init:
      | munge_init(gcb, ...
      |     'divisions', divisions, ...
      |     'div_size', div_size, ...
      |     'order', order, ...
      |     'arith_type_out', arith_type_out, ...
      |     'bin_pt_out', bin_pt_out);
      settings: AttributesFormatString=|
      | split:[1 32 32 32 32 32 32 32 32]
      | join:[0 8 0 7 0 6 0 5 0 4 0 3 0 2 0 1]
      | Unsigned [264,0]
      mask TypeOptions arith_type_out: Unsigned | Signed  (2's comp) | Floating-point
  munge1 : Subsystem  AncestorBlock=casper_library_flow_control/munge  mask(munge){divisions=2^(n_bits_output_words+1), div_size=reshape([ones(1, 2^n_bits_output_words); repmat(n_bits_data, 1 ,2^n_bits_output_words)], 1, 2^(n_bits_output_words+1)), order=[[0:2:2^(n_bits_output_words+1)-2], [1:2:2^(n_bits_output_words+1)-1]], arith_type_out=Unsigned, bin_pt_out=0}
      mask prompts: divisions "Number of divisions"; div_size "Division size (bits)"; order "Division packing order"; arith_type_out "Output arithmetic type"; bin_pt_out "Output binary point"
      mask help: Splits an input bus into the specified number of divisions and then recombines them in the order specified (most significant division = 0,least = number divisions-1)
      mask init:
      | munge_init(gcb, ...
      |     'divisions', divisions, ...
      |     'div_size', div_size, ...
      |     'order', order, ...
      |     'arith_type_out', arith_type_out, ...
      |     'bin_pt_out', bin_pt_out);
      settings: AttributesFormatString=|
      | split:[1 32]
      | join:[0 1]
      | Unsigned [33,0]
      mask TypeOptions arith_type_out: Unsigned | Signed  (2's comp) | Floating-point
  output_control : Subsystem
  time_check : xbsIndex_r4/Assert  assert_type=on  type_source=Explicitly  gui_display_data_type=Fixed-point  arith_type=Unsigned  n_bits=n_bits_timestamp  bin_pt=0  preci_type=Single  exp_width=8  frac_width=24  assert_rate=off  rate_source=Explicitly  period=1  output_port=on  block_type=assert
  time_freq_unpack : Subsystem
  sync_out : Outport
  data_out : Outport  Port=2
  valid_out : Outport  Port=3
  time_out : Outport  Port=4
  freq_out : Outport  Port=5
  recvd : Outport  Port=6
  packet_discarded : Outport  Port=7
  mcnt_timeout : Outport  Port=8
  wires:
  time_freq_unpack/2(freq) -> freq_out/1
  time_freq_unpack/1(time) -> time_out/1
  freq/1 -> freq_check/1
  Constant1/1 -> input_control/7(n_src)
  Constant3/1 -> input_control/6(pkt_size)
  output_control/4(rd_timefreq) -> Delay1/1
  input_control/1(maxcnt) -> output_control/1(maxcnt)
  input_control/3(wr_data) -> Delay23/1
  output_control/1(gen_sync) -> Delay20/1
  data_buffer/1 -> munge1/1(din)
  data_buffer/2 -> Terminator1/1
  output_control/2(rd_en) -> data_buffer/3, Delay21/1
  input_control/2(wr_addr) -> Delay24/1
  input_control/4(we) -> Delay25/1
  board_id/1 -> time_freq_unpack/2(xeng_id)
  din/1 -> data_check/1
  ant/1 -> ant_check/1
  Concat2/1 -> input_control/4(time_freq)
  Constant2/1 -> Concat/1
  Concat/1 -> munge/1(din)
  Delay23/1 -> Concat/2
  input_control/5(discarding) -> packet_discarded/1
  munge/1(dout) -> data_buffer/5
  Constant4/1 -> Concat1/2
  Constant/1 -> Concat1/1
  bus_replicate/1(out) -> data_buffer/2
  Concat1/1 -> bus_replicate/1(in)
  time/1 -> time_check/1
  bus_expand/2(lsb_out1) -> data_out/1
  time_check/1 -> Concat2/1
  freq_check/1 -> Concat2/2
  bus_expand/1(msb_out2) -> Logical/2
  Logical/1 -> recvd/1
  input_control/6(mcnt_timeout) -> mcnt_timeout/1
  data_check/1 -> input_control/1(data_in)
  valid_in/1 -> input_control/2(valid)
  pkt_idx/1 -> input_control/3(pkt_idx)
  ant_check/1 -> input_control/5(src)
  Delay20/1 -> sync_out/1
  Delay21/1 -> Logical/1, valid_out/1
  Delay1/1 -> time_freq_unpack/1(din)
  munge1/1(dout) -> bus_expand/1(bus_in)
  Delay25/1 -> data_buffer/6
  output_control/3(rd_addr) -> data_buffer/1
  Delay24/1 -> data_buffer/4

== system s_b16a4x512f/sys2/pre_process ==
  data_in : Inport
  valid_in : Inport  Port=2
  eof_in : Inport  Port=3
  spead_time48 : Inport  Port=4
  spead_fengid : Inport  Port=5
  dest_xeng : Inport  Port=6
  this_xeng_id : Inport  Port=7
  freq_in : Inport  Port=8
  Delay{3..5,7,9..10} (6 alike) : xbsIndex_r4/Delay  rst=off  infoeditControl=Selection of Reset will increase slice count due to use of real FFs and instead of SRLs  en=off  latency=1  reg_retiming=on  dbl_ovrd=off  block_type=delay
      settings: xl_area=[0, 0, 0, 0, 0, 0, 0]
  Logical3 : xbsIndex_r4/Logical  logical_function=AND  inputs=2  en=off  latency=0  precision=Full  arith_type=Unsigned  n_bits=8  bin_pt=2  align_bp=on  dbl_ovrd=off  block_type=logical
      settings: xl_area=[0, 0, 0, 0, 0, 0, 0]
  correct_xengine : xbsIndex_r4/Relational  mode=a=b  op_type=Bool  en=off  latency=1  dbl_ovrd=off  block_type=relational
      settings: xl_area=[0, 0, 0, 0, 0, 0, 0]  block_version=10.1.3
  xeng : xbsIndex_r4/Slice  nbits=share_bits  boolean_output=off  mode=Lower Bit Location + Width  bit1=0  base1=MSB of Input  bit0=0  base0=LSB of Input  dbl_ovrd=off  block_type=slice
      settings: block_version=10.1.3
  data_out : Outport
  valid : Outport  Port=2
  eof_out : Outport  Port=3
  timestamp : Outport  Port=4
  feng_id : Outport  Port=5
  freq_out : Outport  Port=6
  wires:
  Delay3/1 -> Logical3/1
  this_xeng_id/1 -> xeng/1
  Logical3/1 -> valid/1
  valid_in/1 -> Delay3/1
  xeng/1 -> correct_xengine/2
  eof_in/1 -> Delay7/1
  data_in/1 -> Delay5/1
  Delay5/1 -> data_out/1
  Delay4/1 -> freq_out/1
  Delay7/1 -> eof_out/1
  Delay9/1 -> timestamp/1
  Delay10/1 -> feng_id/1
  freq_in/1 -> Delay4/1
  spead_fengid/1 -> Delay10/1
  correct_xengine/1 -> Logical3/2
  spead_time48/1 -> Delay9/1
  dest_xeng/1 -> correct_xengine/1
